simulink model "codeur_registre"  (R2023b)
settings: Solver=FixedStepDiscrete  StartTime=0.0  StopTime=Tstop  FixedStep=1  RelTol=1e-3
libraries: simulink x1
settings Model: Creator=e2604176  LastModifiedBy=e2604176
settings OptimizationCC: BooleanDataType=off

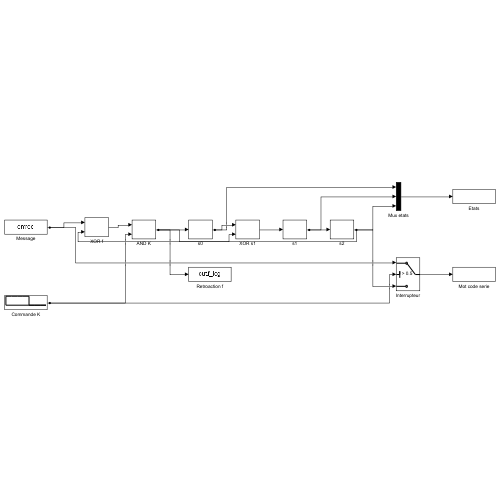
[thumbnail: Simulink's stored preview of the top-level diagram]
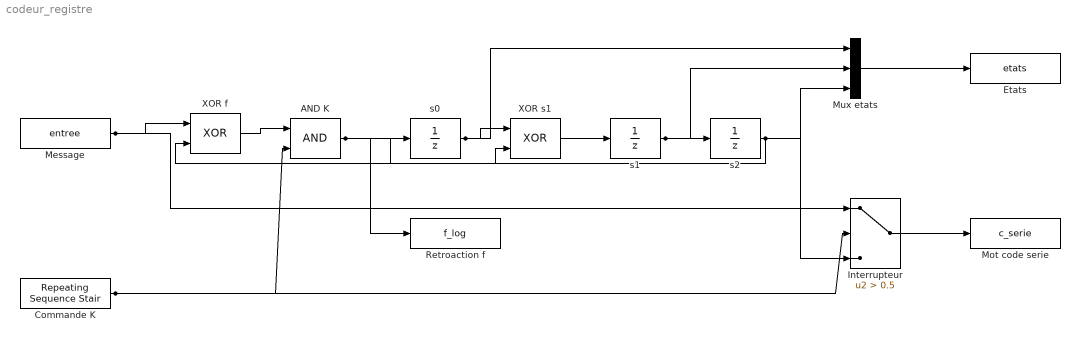
== system codeur_registre ==
  AND K : Logic  AllPortsSameDT=off  OutDataTypeStr=boolean
  Commande K : simulink/Sources/Repeating Sequence Stair  OutValues=[1 1 1 1 0 0 0]  tsamp=1  OutMin=[]  OutMax=[]  OutDataTypeStr=double  OutputDataTypeScalingMode=double  OutDataType=fixdt(0,8)  ConRadixGroup=Best Precision: Vector-wise  OutScaling=2^-12
  Etats : ToWorkspace  VariableName=etats  SampleTime=-1
  Interrupteur : Switch  Criteria=u2 > Threshold  Threshold=0.5  SaturateOnIntegerOverflow=off  InputSameDT=off
  Message : FromWorkspace  VariableName=entree  SampleTime=1  Interpolate=off  OutputAfterFinalValue=Setting to zero
  Mot code serie : ToWorkspace  VariableName=c_serie  SampleTime=-1
  Mux etats : Mux  Inputs=3
  Retroaction f : ToWorkspace  VariableName=f_log  SampleTime=-1
  XOR f : Logic  Operator=XOR  AllPortsSameDT=off  OutDataTypeStr=boolean
  XOR s1 : Logic  Operator=XOR  AllPortsSameDT=off  OutDataTypeStr=boolean
  s0 : UnitDelay  SampleTime=-1  HasFrameUpgradeWarning=on
  s1 : UnitDelay  SampleTime=-1  HasFrameUpgradeWarning=on
  s2 : UnitDelay  SampleTime=-1  HasFrameUpgradeWarning=on
  wires:
  Message/1 -> XOR f/1, Interrupteur/1
  s2/1 -> XOR f/2, Interrupteur/3, Mux etats/3
  XOR f/1 -> AND K/1
  Commande K/1 -> AND K/2, Interrupteur/2
  AND K/1 -> s0/1, XOR s1/2, Retroaction f/1
  s0/1 -> XOR s1/1, Mux etats/1
  XOR s1/1 -> s1/1
  s1/1 -> s2/1, Mux etats/2
  Interrupteur/1 -> Mot code serie/1
  Mux etats/1 -> Etats/1
